simulink model "AXU5EV_RealIO_NoPower"  (R2026b)
settings: Solver=FixedStepDiscrete  StopTime=4e-4  FixedStep=2e-8
settings Model: Creator=lww  LastModifiedBy=lww

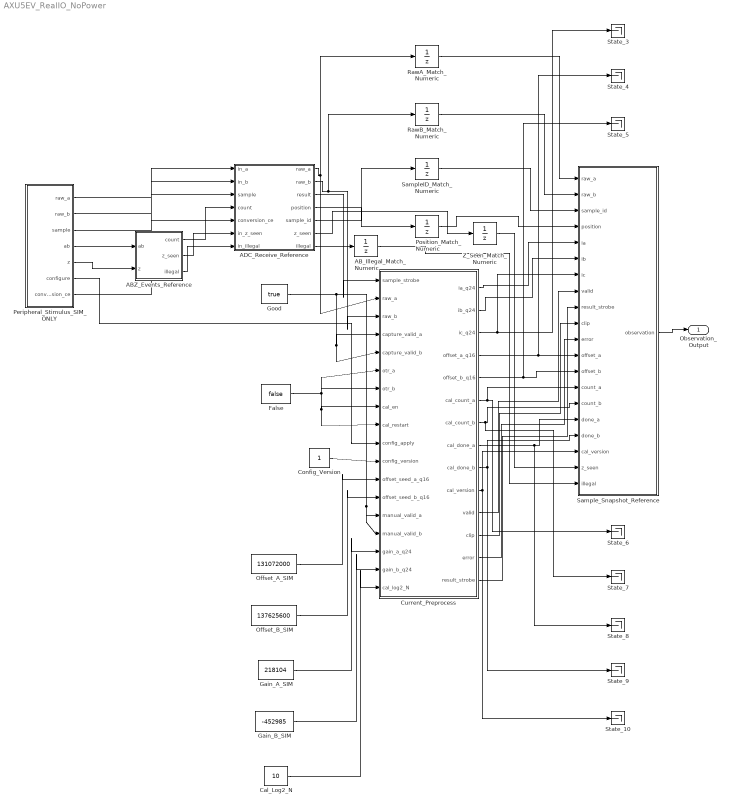
== system AXU5EV_RealIO_NoPower ==
  ABZ_Events_Reference : MATLAB Function  TreatAsAtomicUnit=on
  AB_Illegal_Match_Numeric : UnitDelay  SampleTime=-1
  ADC_Receive_Reference : MATLAB Function  TreatAsAtomicUnit=on
  Cal_Log2_N : Constant  Value=10  OutDataTypeStr=uint8
  Config_Version : Constant  OutDataTypeStr=uint32
  Current_Preprocess : Subsystem
  False : Constant  Value=false  OutDataTypeStr=boolean
  Gain_A_SIM : Constant  Value=218104  OutDataTypeStr=int32
  Gain_B_SIM : Constant  Value=-452985  OutDataTypeStr=int32
  Good : Constant  Value=true  OutDataTypeStr=boolean
  Offset_A_SIM : Constant  Value=131072000  OutDataTypeStr=int32
  Offset_B_SIM : Constant  Value=137625600  OutDataTypeStr=int32
  Peripheral_Stimulus_SIM_ONLY : MATLAB Function  TreatAsAtomicUnit=on
  Position_Match_Numeric : UnitDelay  SampleTime=-1
  RawA_Match_Numeric : UnitDelay  SampleTime=-1
  RawB_Match_Numeric : UnitDelay  SampleTime=-1
  SampleID_Match_Numeric : UnitDelay  SampleTime=-1
  Sample_Snapshot_Reference : MATLAB Function  TreatAsAtomicUnit=on
  State_{3..10} (8 alike) : Terminator
  Z_Seen_Match_Numeric : UnitDelay  SampleTime=-1
  Observation_Output : Outport  OutDataTypeStr=int64
  wires:
  ADC_Receive_Reference/5(sample_id) -> SampleID_Match_Numeric/1
  ADC_Receive_Reference/4(position) -> Position_Match_Numeric/1
  Cal_Log2_N/1 -> Current_Preprocess/18(cal_log2_N)
  Gain_B_SIM/1 -> Current_Preprocess/17(gain_b_q24)
  Gain_A_SIM/1 -> Current_Preprocess/16(gain_a_q24)
  Offset_B_SIM/1 -> Current_Preprocess/13(offset_seed_b_q16)
  Offset_A_SIM/1 -> Current_Preprocess/12(offset_seed_a_q16)
  Config_Version/1 -> Current_Preprocess/11(config_version)
  Peripheral_Stimulus_SIM_ONLY/6(configure) -> Current_Preprocess/10(config_apply)
  False/1 -> Current_Preprocess/9(cal_restart), Current_Preprocess/8(cal_en), Current_Preprocess/6(otr_a), Current_Preprocess/7(otr_b)
  Good/1 -> Current_Preprocess/4(capture_valid_a), Current_Preprocess/5(capture_valid_b), Current_Preprocess/15(manual_valid_b), Current_Preprocess/14(manual_valid_a)
  ADC_Receive_Reference/2(raw_b) -> Current_Preprocess/3(raw_b), RawB_Match_Numeric/1
  ADC_Receive_Reference/1(raw_a) -> Current_Preprocess/2(raw_a), RawA_Match_Numeric/1
  ADC_Receive_Reference/3(result) -> Current_Preprocess/1(sample_strobe)
  Peripheral_Stimulus_SIM_ONLY/7(conversion_ce) -> ADC_Receive_Reference/5(conversion_ce)
  ABZ_Events_Reference/1(count) -> ADC_Receive_Reference/4(count)
  Peripheral_Stimulus_SIM_ONLY/5(z) -> ABZ_Events_Reference/2(z)
  Peripheral_Stimulus_SIM_ONLY/4(ab) -> ABZ_Events_Reference/1(ab)
  Peripheral_Stimulus_SIM_ONLY/3(sample) -> ADC_Receive_Reference/3(sample)
  Peripheral_Stimulus_SIM_ONLY/2(raw_b) -> ADC_Receive_Reference/2(in_b)
  Peripheral_Stimulus_SIM_ONLY/1(raw_a) -> ADC_Receive_Reference/1(in_a)
  ABZ_Events_Reference/2(z_seen) -> ADC_Receive_Reference/6(in_z_seen)
  ABZ_Events_Reference/3(illegal) -> ADC_Receive_Reference/7(in_illegal)
  AB_Illegal_Match_Numeric/1 -> Sample_Snapshot_Reference/20(illegal)
  Z_Seen_Match_Numeric/1 -> Sample_Snapshot_Reference/19(z_seen)
  ADC_Receive_Reference/7(illegal) -> AB_Illegal_Match_Numeric/1
  ADC_Receive_Reference/6(z_seen) -> Z_Seen_Match_Numeric/1
  RawA_Match_Numeric/1 -> Sample_Snapshot_Reference/1(raw_a)
  RawB_Match_Numeric/1 -> Sample_Snapshot_Reference/2(raw_b)
  SampleID_Match_Numeric/1 -> Sample_Snapshot_Reference/3(sample_id)
  Position_Match_Numeric/1 -> Sample_Snapshot_Reference/4(position)
  Current_Preprocess/1(ia_q24) -> Sample_Snapshot_Reference/5(ia)
  Current_Preprocess/2(ib_q24) -> Sample_Snapshot_Reference/6(ib)
  Current_Preprocess/3(ic_q24) -> State_3/1, Sample_Snapshot_Reference/7(ic)
  Current_Preprocess/11(valid) -> Sample_Snapshot_Reference/8(valid)
  Current_Preprocess/14(result_strobe) -> Sample_Snapshot_Reference/9(result_strobe)
  Current_Preprocess/12(clip) -> Sample_Snapshot_Reference/10(clip)
  Current_Preprocess/13(error) -> Sample_Snapshot_Reference/11(error)
  Current_Preprocess/4(offset_a_q16) -> State_4/1, Sample_Snapshot_Reference/12(offset_a)
  Current_Preprocess/5(offset_b_q16) -> State_5/1, Sample_Snapshot_Reference/13(offset_b)
  Current_Preprocess/6(cal_count_a) -> State_6/1, Sample_Snapshot_Reference/14(count_a)
  Current_Preprocess/7(cal_count_b) -> State_7/1, Sample_Snapshot_Reference/15(count_b)
  Current_Preprocess/8(cal_done_a) -> State_8/1, Sample_Snapshot_Reference/16(done_a)
  Current_Preprocess/9(cal_done_b) -> State_9/1, Sample_Snapshot_Reference/17(done_b)
  Current_Preprocess/10(cal_version) -> State_10/1, Sample_Snapshot_Reference/18(cal_version)
  Sample_Snapshot_Reference/1(observation) -> Observation_Output/1

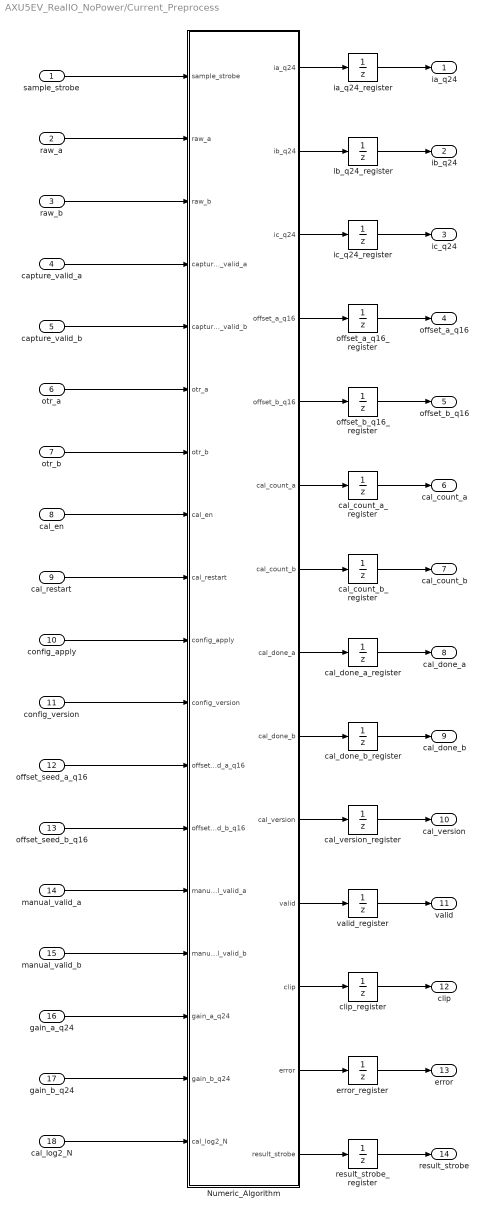
== system AXU5EV_RealIO_NoPower/Current_Preprocess ==
  sample_strobe : Inport  OutDataTypeStr=boolean  SampleTime=2e-8
  raw_a : Inport  Port=2  OutDataTypeStr=uint16  SampleTime=2e-8
  raw_b : Inport  Port=3  OutDataTypeStr=uint16  SampleTime=2e-8
  capture_valid_a : Inport  Port=4  OutDataTypeStr=boolean  SampleTime=2e-8
  capture_valid_b : Inport  Port=5  OutDataTypeStr=boolean  SampleTime=2e-8
  otr_a : Inport  Port=6  OutDataTypeStr=boolean  SampleTime=2e-8
  otr_b : Inport  Port=7  OutDataTypeStr=boolean  SampleTime=2e-8
  cal_en : Inport  Port=8  OutDataTypeStr=boolean  SampleTime=2e-8
  cal_restart : Inport  Port=9  OutDataTypeStr=boolean  SampleTime=2e-8
  config_apply : Inport  Port=10  OutDataTypeStr=boolean  SampleTime=2e-8
  config_version : Inport  Port=11  OutDataTypeStr=uint32  SampleTime=2e-8
  offset_seed_a_q16 : Inport  Port=12  OutDataTypeStr=int32  SampleTime=2e-8
  offset_seed_b_q16 : Inport  Port=13  OutDataTypeStr=int32  SampleTime=2e-8
  manual_valid_a : Inport  Port=14  OutDataTypeStr=boolean  SampleTime=2e-8
  manual_valid_b : Inport  Port=15  OutDataTypeStr=boolean  SampleTime=2e-8
  gain_a_q24 : Inport  Port=16  OutDataTypeStr=int32  SampleTime=2e-8
  gain_b_q24 : Inport  Port=17  OutDataTypeStr=int32  SampleTime=2e-8
  cal_log2_N : Inport  Port=18  OutDataTypeStr=uint8  SampleTime=2e-8
  Numeric_Algorithm : MATLAB Function  TreatAsAtomicUnit=on
  cal_count_a_register : UnitDelay  SampleTime=-1
  cal_count_b_register : UnitDelay  SampleTime=-1
  cal_done_a_register : UnitDelay  SampleTime=-1
  cal_done_b_register : UnitDelay  SampleTime=-1
  cal_version_register : UnitDelay  SampleTime=-1
  clip_register : UnitDelay  SampleTime=-1
  error_register : UnitDelay  SampleTime=-1
  ia_q24_register : UnitDelay  SampleTime=-1
  ib_q24_register : UnitDelay  SampleTime=-1
  ic_q24_register : UnitDelay  SampleTime=-1
  offset_a_q16_register : UnitDelay  SampleTime=-1
  offset_b_q16_register : UnitDelay  SampleTime=-1
  result_strobe_register : UnitDelay  SampleTime=-1
  valid_register : UnitDelay  SampleTime=-1
  ia_q24 : Outport  OutDataTypeStr=int32
  ib_q24 : Outport  Port=2  OutDataTypeStr=int32
  ic_q24 : Outport  Port=3  OutDataTypeStr=int32
  offset_a_q16 : Outport  Port=4  OutDataTypeStr=int32
  offset_b_q16 : Outport  Port=5  OutDataTypeStr=int32
  cal_count_a : Outport  Port=6  OutDataTypeStr=uint16
  cal_count_b : Outport  Port=7  OutDataTypeStr=uint16
  cal_done_a : Outport  Port=8  OutDataTypeStr=boolean
  cal_done_b : Outport  Port=9  OutDataTypeStr=boolean
  cal_version : Outport  Port=10  OutDataTypeStr=uint32
  valid : Outport  Port=11  OutDataTypeStr=boolean
  clip : Outport  Port=12  OutDataTypeStr=boolean
  error : Outport  Port=13  OutDataTypeStr=uint16
  result_strobe : Outport  Port=14  OutDataTypeStr=boolean
  wires:
  Numeric_Algorithm/14(result_strobe) -> result_strobe_register/1
  Numeric_Algorithm/13(error) -> error_register/1
  Numeric_Algorithm/12(clip) -> clip_register/1
  Numeric_Algorithm/11(valid) -> valid_register/1
  Numeric_Algorithm/10(cal_version) -> cal_version_register/1
  Numeric_Algorithm/9(cal_done_b) -> cal_done_b_register/1
  Numeric_Algorithm/8(cal_done_a) -> cal_done_a_register/1
  Numeric_Algorithm/7(cal_count_b) -> cal_count_b_register/1
  Numeric_Algorithm/6(cal_count_a) -> cal_count_a_register/1
  Numeric_Algorithm/5(offset_b_q16) -> offset_b_q16_register/1
  Numeric_Algorithm/4(offset_a_q16) -> offset_a_q16_register/1
  Numeric_Algorithm/3(ic_q24) -> ic_q24_register/1
  Numeric_Algorithm/2(ib_q24) -> ib_q24_register/1
  cal_log2_N/1 -> Numeric_Algorithm/18(cal_log2_N)
  gain_b_q24/1 -> Numeric_Algorithm/17(gain_b_q24)
  gain_a_q24/1 -> Numeric_Algorithm/16(gain_a_q24)
  manual_valid_b/1 -> Numeric_Algorithm/15(manual_valid_b)
  manual_valid_a/1 -> Numeric_Algorithm/14(manual_valid_a)
  offset_seed_b_q16/1 -> Numeric_Algorithm/13(offset_seed_b_q16)
  offset_seed_a_q16/1 -> Numeric_Algorithm/12(offset_seed_a_q16)
  config_version/1 -> Numeric_Algorithm/11(config_version)
  config_apply/1 -> Numeric_Algorithm/10(config_apply)
  cal_restart/1 -> Numeric_Algorithm/9(cal_restart)
  cal_en/1 -> Numeric_Algorithm/8(cal_en)
  otr_b/1 -> Numeric_Algorithm/7(otr_b)
  otr_a/1 -> Numeric_Algorithm/6(otr_a)
  capture_valid_b/1 -> Numeric_Algorithm/5(capture_valid_b)
  capture_valid_a/1 -> Numeric_Algorithm/4(capture_valid_a)
  raw_b/1 -> Numeric_Algorithm/3(raw_b)
  raw_a/1 -> Numeric_Algorithm/2(raw_a)
  sample_strobe/1 -> Numeric_Algorithm/1(sample_strobe)
  Numeric_Algorithm/1(ia_q24) -> ia_q24_register/1
  ia_q24_register/1 -> ia_q24/1
  ib_q24_register/1 -> ib_q24/1
  ic_q24_register/1 -> ic_q24/1
  offset_a_q16_register/1 -> offset_a_q16/1
  offset_b_q16_register/1 -> offset_b_q16/1
  cal_count_a_register/1 -> cal_count_a/1
  cal_count_b_register/1 -> cal_count_b/1
  cal_done_a_register/1 -> cal_done_a/1
  cal_done_b_register/1 -> cal_done_b/1
  cal_version_register/1 -> cal_version/1
  valid_register/1 -> valid/1
  clip_register/1 -> clip/1
  error_register/1 -> error/1
  result_strobe_register/1 -> result_strobe/1

== matlab function AXU5EV_RealIO_NoPower/Current_Preprocess/Numeric_Algorithm ==
  data: sample_strobe input; ia_q24 output; raw_a input; raw_b input; capture_valid_a input; capture_valid_b input; otr_a input; otr_b input; cal_en input; cal_restart input; config_apply input; config_version input; offset_seed_a_q16 input; offset_seed_b_q16 input; manual_valid_a input; manual_valid_b input; gain_a_q24 input; gain_b_q24 input; cal_log2_N input; ib_q24 output; ic_q24 output; offset_a_q16 output; offset_b_q16 output; cal_count_a output; cal_count_b output; cal_done_a output; cal_done_b output; cal_version output; valid output; clip output; error output; result_strobe output
function [ia_q24,ib_q24,ic_q24,offset_a_q16,offset_b_q16,cal_count_a,cal_count_b,cal_done_a,cal_done_b,cal_version,valid,clip,error,result_strobe] = f(sample_strobe,raw_a,raw_b,capture_valid_a,capture_valid_b,otr_a,otr_b,cal_en,cal_restart,config_apply,config_version,offset_seed_a_q16,offset_seed_b_q16,manual_valid_a,manual_valid_b,gain_a_q24,gain_b_q24,cal_log2_N)
%#codegen
[ia_q24,ib_q24,ic_q24,offset_a_q16,offset_b_q16,cal_count_a,cal_count_b,cal_done_a,cal_done_b,cal_version,valid,clip,error,result_strobe] = ax03b1_current_preprocess(sample_strobe,raw_a,raw_b,capture_valid_a,capture_valid_b,otr_a,otr_b,cal_en,cal_restart,config_apply,config_version,offset_seed_a_q16,offset_seed_b_q16,manual_valid_a,manual_valid_b,gain_a_q24,gain_b_q24,cal_log2_N);
end

== matlab function AXU5EV_RealIO_NoPower/ADC_Receive_Reference ==
  data: in_a input; raw_a output; in_b input; sample input; count input; raw_b output; result output; position output; sample_id output; conversion_ce input; in_z_seen input; in_illegal input; z_seen output; illegal output
function [raw_a,raw_b,result,position,sample_id,z_seen,illegal]=f(in_a,in_b,sample,count,conversion_ce,in_z_seen,in_illegal)
%#codegen
[raw_a,raw_b,result,position,sample_id,z_seen,illegal]=ax03b1_adc_reference(in_a,in_b,sample,count,conversion_ce,in_z_seen,in_illegal);
end

== matlab function AXU5EV_RealIO_NoPower/Peripheral_Stimulus_SIM_ONLY ==
  settings: updateMethod=DISCRETE  sampleTime=2e-8
  data: raw_a output; raw_b output; sample output; ab output; z output; configure output; conversion_ce output
function [raw_a,raw_b,sample,ab,z,configure,conversion_ce]=f()
%#codegen
[raw_a,raw_b,sample,ab,z,configure,conversion_ce]=ax03b1_stimulus();
end

== matlab function AXU5EV_RealIO_NoPower/ABZ_Events_Reference ==
  data: ab input; count output; z input; z_seen output; illegal output
function [count,z_seen,illegal] = f(ab,z)
%#codegen
[count,z_seen,illegal] = ax03b1_abz_reference(ab,z);
end

== matlab function AXU5EV_RealIO_NoPower/Sample_Snapshot_Reference ==
  data: raw_a input; observation output; raw_b input; sample_id input; position input; ia input; ib input; ic input; valid input; result_strobe input; clip input; error input; offset_a input; offset_b input; count_a input; count_b input; done_a input; done_b input; cal_version input; z_seen input; illegal input
function observation=f(raw_a,raw_b,sample_id,position,ia,ib,ic,valid,result_strobe,clip,error,offset_a,offset_b,count_a,count_b,done_a,done_b,cal_version,z_seen,illegal)
%#codegen
observation=ax03b1_snapshot_reference(raw_a,raw_b,sample_id,position,ia,ib,ic,valid,result_strobe,clip,error,offset_a,offset_b,count_a,count_b,done_a,done_b,cal_version,z_seen,illegal);
end
